simulink model "noslip_softsoil"  (R2022b)
settings: Solver=VariableStepAuto  StartTime=0.0  StopTime=10.0  RelTol=1e-3
settings Model: Creator=22872  LastModifiedBy=22872

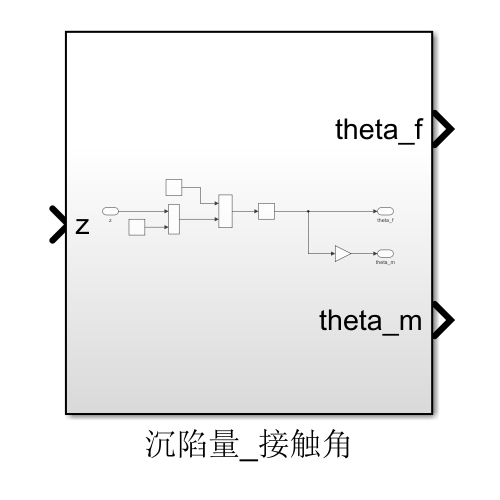
[thumbnail: Simulink's stored preview of the top-level diagram]
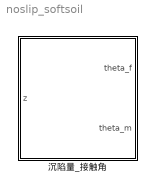
== system noslip_softsoil ==
  沉陷量_接触角 : Subsystem

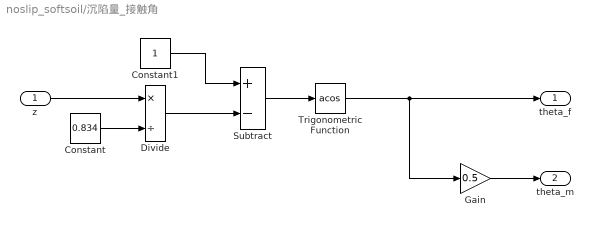
== system noslip_softsoil/沉陷量_接触角 ==
  z : Inport
  Constant : Constant  Value=0.834
  Constant1 : Constant
  Divide : Product  Inputs=*/
  Gain : Gain  Gain=0.5
  Subtract : Sum  Inputs=+-
  Trigonometric Function : Trigonometry  Operator=acos
  theta_f : Outport
  theta_m : Outport  Port=2
  wires:
  z/1 -> Divide/1
  Constant/1 -> Divide/2
  Divide/1 -> Subtract/2
  Constant1/1 -> Subtract/1
  Subtract/1 -> Trigonometric Function/1
  Trigonometric Function/1 -> Gain/1, theta_f/1
  Gain/1 -> theta_m/1
